simulink model "step6_motor_simulink"  (R2026b)
settings: Solver=VariableStepAuto  StopTime=30
PreLoadFcn:
  | params
values from neighbouring files (symbols this model uses):
  b = 1e-8    (= 1e-08)    [params.m]
  J = 1.06e-6    (= 1.06e-06)    [params.m]
  Ke = 0.0025    [params.m]
  Kt = 0.0025    [params.m]
  L = 1e-3    (= 0.001)    [params.m]
  R = 30    [params.m]
settings Model: Creator=nkech  LastModifiedBy=nkech

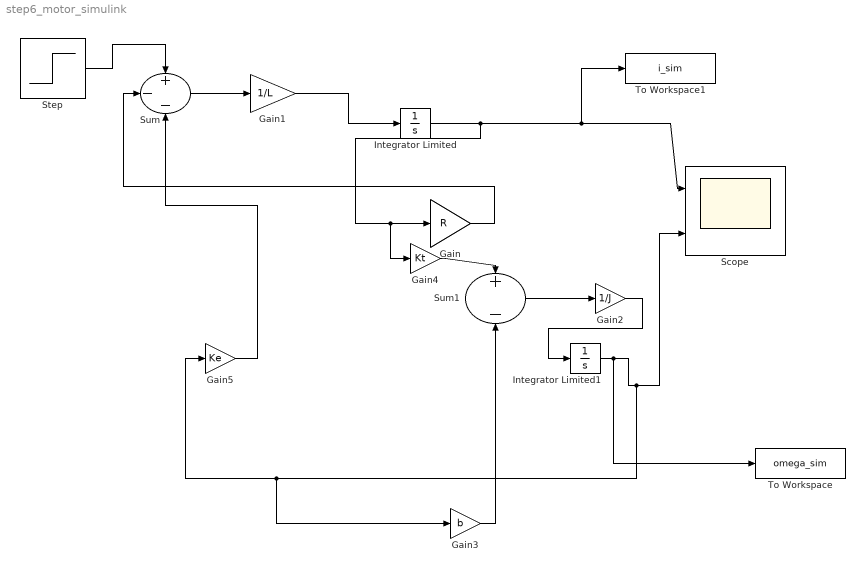
== system step6_motor_simulink ==
  Gain : Gain  Gain=R
  Gain1 : Gain  Gain=1/L
  Gain2 : Gain  Gain=1/J
  Gain3 : Gain  Gain=b
  Gain4 : Gain  Gain=Kt
  Gain5 : Gain  Gain=Ke
  Integrator Limited : Integrator  UpperSaturationLimit=1  LowerSaturationLimit=0
  Integrator Limited1 : Integrator  UpperSaturationLimit=1  LowerSaturationLimit=0
  Scope : Scope  NumInputPorts=2
      settings: ActiveDisplayYMinimum=-0.6154434661543704  ActiveDisplayYMaximum=0.50574858939462408
  Step : Step  Time=0  FinalValue=V  SampleTime=0
  Sum : Sum  Inputs=+--
  Sum1 : Sum  Inputs=+-
  To Workspace : ToWorkspace  VariableName=omega_sim  SaveFormat=Timeseries  SampleTime=-1
  To Workspace1 : ToWorkspace  VariableName=i_sim  SaveFormat=Timeseries  SampleTime=-1
  wires:
  Sum/1 -> Gain1/1
  Gain1/1 -> Integrator Limited/1
  Gain/1 -> Sum/2
  Integrator Limited/1 -> Gain/1, Gain4/1, To Workspace1/1, Scope/1
  Gain4/1 -> Sum1/1
  Sum1/1 -> Gain2/1
  Gain2/1 -> Integrator Limited1/1
  Integrator Limited1/1 -> To Workspace/1, Gain5/1, Gain3/1, Scope/2
  Gain3/1 -> Sum1/2
  Gain5/1 -> Sum/3
  Step/1 -> Sum/1
